simulink model "mpc_psm"  (R2026b)
settings: Solver=ode23tb  StopTime=param.sim.simlength  FixedStep=param.glb_time.tc  MaxStep=param.glb_time.tc
values from neighbouring files (symbols this model uses):
  param = struct()    [init_model.m]
undefined symbols (not defined in the file or in its folder): tc
libraries: fl_lib x28, nesl_utility x13, cstblocks_lti x6, lithium_ion_battery x1, dclink_with_center_tap x1, ideal_bridges_lib x1, dead_time_generator_cmos_simulink x1, single_phase_pwm_modulator x1, threephase_inductor_lib x1, simple_flexible_shaft x1, permanent_magnet_synchronous_machine x1
(part 3 of 3)

== system mpc_psm/inv_psm_mod1/inverter_ctrl/inverter_control/phase_compensation_1/alignment_ctrl/pi ==
  u_ref : Inport
  u : Inport  Port=2
  1/Ti : Gain  Gain=kp  SaturateOnIntegerOverflow=on  OutDataTypeStr=Inherit: Same as input  ParamDataTypeStr=Inherit: Same as input
  Saturation : Saturate  UpperLimit=lim_up  LowerLimit=lim_down
  Sum1 : Sum  Inputs=+++  SaturateOnIntegerOverflow=on
  Sum2 : Sum  Inputs=-+  SaturateOnIntegerOverflow=on
  Sum3 : Sum  Inputs=-+  SaturateOnIntegerOverflow=on
  Unit Delay4 : UnitDelay  SampleTime=-1
  kp : Gain  Gain=ki  SaturateOnIntegerOverflow=on  OutDataTypeStr=Inherit: Same as input  ParamDataTypeStr=Inherit: Same as input
  y : Outport
  wires:
  1/Ti/1 -> Sum1/1, Sum3/1
  kp/1 -> Sum1/2
  Sum3/1 -> Unit Delay4/1
  Unit Delay4/1 -> Sum1/3
  u_ref/1 -> Sum2/2
  u/1 -> Sum2/1
  Sum2/1 -> kp/1, 1/Ti/1
  Sum1/1 -> Saturation/1
  Saturation/1 -> Sum3/2, y/1

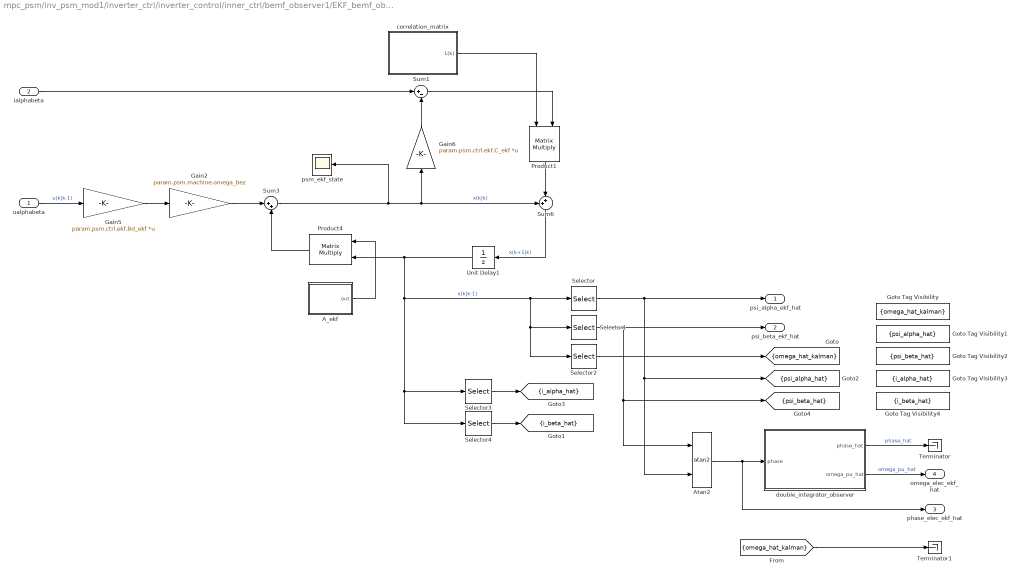
== system mpc_psm/inv_psm_mod1/inverter_ctrl/inverter_control/inner_ctrl/bemf_observer1/EKF_bemf_observer/extended_kalman_observer ==
  ualphabeta : Inport
  ialphabeta : Inport  Port=2
  A_ekf : Subsystem
  Atan2 : Trigonometry  Operator=atan2
  Gain2 : Gain  Gain=param.psm.machine.omega_bez
  Gain5 : Gain  Gain=param.psm.ctrl.ekf.Bd_ekf  Multiplication=Matrix(K*u)
  Gain6 : Gain  Gain=param.psm.ctrl.ekf.C_ekf  Multiplication=Matrix(K*u)
  Goto Tag Visibility : GotoTagVisibility  GotoTag=omega_hat_kalman
  Goto Tag Visibility1 : GotoTagVisibility  GotoTag=psi_alpha_hat
  Goto Tag Visibility2 : GotoTagVisibility  GotoTag=psi_beta_hat
  Goto Tag Visibility3 : GotoTagVisibility  GotoTag=i_alpha_hat
  Goto Tag Visibility4 : GotoTagVisibility  GotoTag=i_beta_hat
  Product1 : Product  Multiplication=Matrix(*)
  Product4 : Product  Multiplication=Matrix(*)
  Selector : Selector  InputPortWidth=6  IndexOptions=Index vector (dialog)  Indices=3  OutputSizes=1  RuntimeRangeChecks=off
  Selector1 : Selector  InputPortWidth=6  IndexOptions=Index vector (dialog)  Indices=4  OutputSizes=1  RuntimeRangeChecks=off
  Selector2 : Selector  InputPortWidth=6  IndexOptions=Index vector (dialog)  Indices=5  OutputSizes=1  RuntimeRangeChecks=off
  Selector3 : Selector  InputPortWidth=6  IndexOptions=Index vector (dialog)  Indices=1  OutputSizes=1  RuntimeRangeChecks=off
  Selector4 : Selector  InputPortWidth=6  IndexOptions=Index vector (dialog)  Indices=2  OutputSizes=1  RuntimeRangeChecks=off
  Sum1 : Sum  Inputs=|+-
  Sum3 : Sum  Inputs=|++
  Sum6 : Sum  Inputs=++|
  Terminator : Terminator
  Terminator1 : Terminator
  Unit Delay1 : UnitDelay  InitialCondition=[0 0 1 1 0 0]*param.glb_time.ts_inv  SampleTime=-1
  correlation_matrix : Subsystem
  double_integrator_observer : Subsystem
  psm_ekf_state : Scope
      settings: ActiveDisplayYMinimum=-2.6651275002473325  ActiveDisplayYMaximum=3.9005956712949552
  psi_alpha_ekf_hat : Outport
  psi_beta_ekf_hat : Outport  Port=2
  phase_elec_ekf_hat : Outport  Port=3
  omega_elec_ekf_hat : Outport  Port=4
  tag scope: i_alpha_hat=scoped, i_beta_hat=scoped, omega_hat_kalman=scoped, psi_alpha_hat=scoped, psi_beta_hat=scoped
  wires:
  Gain5/1 -> Gain2/1
  Gain6/1 -> Sum1/2
  Sum6/1 -> Unit Delay1/1  "x(k+1|k)"
  Sum1/1 -> Product1/2
  ialphabeta/1 -> Sum1/1
  ualphabeta/1 -> Gain5/1  "u(k|k-1)"
  Sum3/1 -> psm_ekf_state/1, Gain6/1, Sum6/1  "x(k|k)"
  Unit Delay1/1 -> Selector2/1, Selector1/1, Selector/1, Selector3/1, Selector4/1, Product4/2  "x(k|k-1)"
  A_ekf/1(out) -> Product4/1
  Selector1/1 -> Atan2/1, [psi_beta_hat], psi_beta_ekf_hat/1
  Selector/1 -> Atan2/2, [psi_alpha_hat], psi_alpha_ekf_hat/1
  Selector2/1 -> [omega_hat_kalman]
  Selector3/1 -> [i_alpha_hat]
  Selector4/1 -> [i_beta_hat]
  Product4/1 -> Sum3/2
  Atan2/1 -> phase_elec_ekf_hat/1, double_integrator_observer/1(phase)
  Gain2/1 -> Sum3/1
  Product1/1 -> Sum6/2
  correlation_matrix/1(L(k)) -> Product1/1
  double_integrator_observer/1(phase_hat) -> Terminator/1  "phase_hat"
  double_integrator_observer/2(omega_pu_hat) -> omega_elec_ekf_hat/1  "omega_pu_hat"
  [omega_hat_kalman] -> Terminator1/1

== system mpc_psm/inv_psm_mod1/inverter_ctrl/inverter_control/inner_ctrl/bemf_observer1/bemf_observer/double_integrator_observer ==
  theta : Inport
  Dead Zone : DeadZone  LowerValue=-0.01  UpperValue=0.01
  Gain : Gain  Gain=param.psm.ctrl.di_obs.komega
  Gain1 : Gain  Gain=param.psm.ctrl.di_obs.ktheta
  Gain2 : Gain  Gain=param.psm.machine.omega_bez
  Gain3 : Gain  Gain=1/param.psm.machine.omega_bez
  Gain4 : Gain  Gain=param.glb_time.ts_inv
  Gain5 : Gain  Gain=param.glb_time.ts_inv
  Gain6 : Gain  Gain=param.glb_time.ts_inv
  Sum : Sum  Inputs=-+|
  Sum1 : Sum  Inputs=|++
  Sum2 : Sum  Inputs=|++
  Sum8 : Sum  Inputs=++|
  Unit Delay1 : UnitDelay  InitialCondition=pi  SampleTime=-1
  Unit Delay2 : UnitDelay  SampleTime=-1
  bounder1 : MATLAB Function  TreatAsAtomicUnit=on
  bounder2 : MATLAB Function  TreatAsAtomicUnit=on
  omega_pu_hat : Outport  VectorParamsAs1DForOutWhenUnconnected=off
  theta_hat : Outport  Port=2  VectorParamsAs1DForOutWhenUnconnected=off
  wires:
  Gain1/1 -> Gain6/1
  theta/1 -> Sum/2  "theta_bemf"
  Sum8/1 -> Unit Delay1/1
  Unit Delay1/1 -> bounder2/1(u)
  Sum1/1 -> Unit Delay2/1
  Gain/1 -> Gain4/1
  Unit Delay2/1 -> omega_pu_hat/1, Sum1/2, Gain5/1
  Sum2/1 -> Sum8/2
  bounder2/1(y) -> Sum2/2, theta_hat/1, Sum/1  "theta_hat"
  bounder1/1(y) -> Gain1/1, Gain/1
  Gain2/1 -> Sum8/1
  Gain3/1 -> Sum1/1
  Gain5/1 -> Gain2/1
  Sum/1 -> bounder1/1(u)
  Gain4/1 -> Gain3/1
  Gain6/1 -> Sum2/1

== system mpc_psm/inv_psm_mod1/inverter_ctrl/inverter_control/inner_ctrl/bemf_observer1/bemf_observer/psi_alpha_hat ==
  ualpha : Inport
  ialpha : Inport  Port=2
  udc : Inport  Port=3
  Gain1 : Gain  Gain=param.psm.ctrl.mpc.R_norm
  Gain2 : Gain  Gain=param.psm.ctrl.emf_fb_p
  Gain3 : Gain  Gain=param.psm.ctrl.emf_p
  Gain4 : Gain  Gain=param.psm.machine.omega_bez
  Gain5 : Gain  Gain=param.psm.ctrl.mpc.L_norm
  Gain6 : Gain  Gain=param.psm.ctrl.u_psm_scale
  Gain7 : Gain  Gain=param.glb_time.ts_inv
  Product : Product  RndMeth=Zero
  Sum : Sum  Inputs=|+-
  Sum1 : Sum  Inputs=|+-
  Sum2 : Sum  Inputs=++-  SaturateOnIntegerOverflow=on
  Sum3 : Sum  Inputs=|++
  Sum4 : Sum  Inputs=+-  SaturateOnIntegerOverflow=on
  Unit Delay1 : UnitDelay  SampleTime=-1
  Unit Delay2 : UnitDelay  SampleTime=-1
  Unit Delay3 : UnitDelay  SampleTime=-1
  psi_s_alpha_hat : Outport  VectorParamsAs1DForOutWhenUnconnected=off
  psi_r_alpha_hat : Outport  Port=2  VectorParamsAs1DForOutWhenUnconnected=off
  wires:
  [psi_r_m_alpha_mod1] -> Sum1/1
  [psi_r_alpha_hat_mod1] -> Sum1/2
  Gain4/1 -> Gain7/1
  Sum2/1 -> Gain4/1
  Gain3/1 -> Sum2/3
  ialpha/1 -> Gain5/1, Gain1/1
  Gain1/1 -> Sum/2
  Sum/1 -> Sum2/2
  ualpha/1 -> Product/1
  Gain5/1 -> Unit Delay3/1
  Unit Delay1/1 -> Sum4/1, psi_s_alpha_hat/1, Gain3/1, Sum3/2
  Sum3/1 -> Unit Delay1/1
  Sum4/1 -> Unit Delay2/1
  Sum1/1 -> Gain2/1
  Gain2/1 -> Sum2/1
  Gain7/1 -> Sum3/1
  Product/1 -> Gain6/1
  Gain6/1 -> Sum/1
  Unit Delay2/1 -> psi_r_alpha_hat/1
  Unit Delay3/1 -> Sum4/2
  udc/1 -> Product/2

== system mpc_psm/inv_psm_mod1/inverter_ctrl/inverter_control/inner_ctrl/bemf_observer1/bemf_observer/psi_beta_hat ==
  ubeta : Inport
  ibeta : Inport  Port=2
  udc : Inport  Port=3
  Gain1 : Gain  Gain=param.psm.ctrl.mpc.R_norm
  Gain2 : Gain  Gain=param.psm.ctrl.emf_fb_p
  Gain3 : Gain  Gain=param.psm.ctrl.emf_p
  Gain4 : Gain  Gain=param.psm.machine.omega_bez
  Gain5 : Gain  Gain=param.psm.ctrl.mpc.L_norm
  Gain6 : Gain  Gain=param.psm.ctrl.u_psm_scale
  Gain7 : Gain  Gain=param.glb_time.ts_inv
  Product : Product  RndMeth=Zero
  Sum : Sum  Inputs=|+-
  Sum1 : Sum  Inputs=|+-
  Sum2 : Sum  Inputs=++-  SaturateOnIntegerOverflow=on
  Sum3 : Sum  Inputs=|++
  Sum4 : Sum  Inputs=+-  SaturateOnIntegerOverflow=on
  Unit Delay1 : UnitDelay  SampleTime=-1
  Unit Delay2 : UnitDelay  SampleTime=-1
  Unit Delay3 : UnitDelay  SampleTime=-1
  psi_s_beta_hat : Outport  VectorParamsAs1DForOutWhenUnconnected=off
  psi_r_beta_hat : Outport  Port=2  VectorParamsAs1DForOutWhenUnconnected=off
  wires:
  Gain5/1 -> Unit Delay3/1
  Sum/1 -> Sum2/2
  Gain1/1 -> Sum/2
  ibeta/1 -> Gain5/1, Gain1/1
  Gain3/1 -> Sum2/3
  Sum2/1 -> Gain4/1
  Gain4/1 -> Gain7/1
  Sum1/1 -> Gain2/1
  [psi_r_beta_hat_mod1] -> Sum1/2
  [psi_r_m_beta_mod1] -> Sum1/1
  Unit Delay1/1 -> Gain3/1, Sum4/1, psi_s_beta_hat/1, Sum3/2
  Sum3/1 -> Unit Delay1/1
  Sum4/1 -> Unit Delay2/1
  Gain2/1 -> Sum2/1
  ubeta/1 -> Product/1
  Gain7/1 -> Sum3/1
  Product/1 -> Gain6/1
  Gain6/1 -> Sum/1
  Unit Delay2/1 -> psi_r_beta_hat/1
  Unit Delay3/1 -> Sum4/2
  udc/1 -> Product/2

== system mpc_psm/inv_psm_mod1/inverter_ctrl/inverter_control/inner_ctrl/bemf_observer1/bemf_observer/theta_bemf_hat ==
  psi_r_alpha_hat : Inport
  psi_r_beta_hat : Inport  Port=2
  Trigonometric Function : Trigonometry  Operator=atan2  OutputSignalType=real
  theta_emf_hat : Outport  VectorParamsAs1DForOutWhenUnconnected=off
  wires:
  psi_r_alpha_hat/1 -> Trigonometric Function/2
  psi_r_beta_hat/1 -> Trigonometric Function/1
  Trigonometric Function/1 -> theta_emf_hat/1

== system mpc_psm/inv_psm_mod1/inverter_ctrl/inverter_control/inner_ctrl/bemf_observer1/bemf_observer_ccaller/Reset Trigger ==
  Step : Step  Time=0.01  InitialValue=1  FinalValue=0
  Out1 : Outport
  wires:
  Step/1 -> Out1/1  "Reset"

== system mpc_psm/inv_psm_mod1/inverter_ctrl/inverter_control/inner_ctrl/bemf_observer1/EKF_bemf_observer/extended_kalman_observer/A_ekf ==
  Gain1 : Gain  Gain=param.psm.ctrl.ekf.A6_pred_ekf
  Gain{7,9..10,13,20} (5 alike) : Gain  Gain=param.psm.machine.omega_bez
  Gain{2,4,6,11,16,18} (6 alike) : Gain  Gain=param.glb_time.ts_inv
  Gain15 : Gain  Gain=param.psm.ctrl.ekf.A2_tilde_ekf
  Gain17 : Gain  Gain=param.psm.ctrl.ekf.A3_tilde_ekf
  Gain3 : Gain  Gain=param.psm.ctrl.ekf.A4_tilde_ekf
  Gain5 : Gain  Gain=param.psm.ctrl.ekf.A5_tilde_ekf
  I1 : Constant  Value=eye(6)
  I2 : Constant  Value=param.psm.ctrl.ekf.A1_tilde_ekf
  Sum7 : Sum  Inputs=+++++++
  out : Outport
  wires:
  Sum7/1 -> out/1
  I2/1 -> Gain11/1
  I1/1 -> Sum7/1
  Gain1/1 -> Gain2/1
  Gain3/1 -> Gain4/1
  Gain5/1 -> Gain6/1
  [omega_hat_kalman] -> Gain1/1
  [psi_alpha_hat] -> Gain3/1
  [psi_beta_hat] -> Gain5/1
  Gain11/1 -> Gain7/1
  Gain4/1 -> Gain9/1
  Gain6/1 -> Gain10/1
  Gain7/1 -> Sum7/2
  Gain9/1 -> Sum7/5
  Gain10/1 -> Sum7/6
  Gain18/1 -> Gain13/1
  Gain16/1 -> Gain20/1
  Gain17/1 -> Gain18/1
  Gain15/1 -> Gain16/1
  Gain13/1 -> Sum7/4
  Gain20/1 -> Sum7/3
  [i_beta_hat] -> Gain17/1
  [i_alpha_hat] -> Gain15/1
  Gain2/1 -> Sum7/7

== system mpc_psm/inv_psm_mod1/inverter_ctrl/inverter_control/inner_ctrl/bemf_observer1/EKF_bemf_observer/extended_kalman_observer/correlation_matrix ==
  A_ekf : Subsystem
  Gain1 : Gain  Gain=param.psm.ctrl.ekf.C_ekf  Multiplication=Matrix(u*K)
  Gain10 : Gain  Gain=param.psm.ctrl.ekf.C_ekf'  Multiplication=Matrix(u*K)
  Gain8 : Gain  Gain=param.psm.ctrl.ekf.C_ekf'  Multiplication=Matrix(u*K)
  Gain9 : Gain  Gain=param.psm.ctrl.ekf.C_ekf  Multiplication=Matrix(K*u)
  I6 : Constant  Value=eye(6)
  Product{,2,5..6} (4 alike) : Product  Multiplication=Matrix(*)
  Product3 : Product  Inputs=*/  Multiplication=Matrix(*)
  Q : Constant  Value=param.psm.ctrl.ekf.Qkalman
  R : Constant  Value=param.psm.ctrl.ekf.Rkalman
  R1 : Constant  Value=eye(2)
  Sum2 : Sum  Inputs=+-|
  Sum4 : Sum  Inputs=|++
  Sum5 : Sum  Inputs=|++
  Transpose : Math  Operator=transpose
  Unit Delay2 : UnitDelay  SampleTime=-1
  L(k) : Outport
  wires:
  A_ekf/1(out) -> Transpose/1, Product5/1
  Product6/1 -> Sum5/1
  Product3/1 -> Product/2
  Gain8/1 -> Product/1
  Sum4/1 -> Product3/2
  Sum5/1 -> Gain8/1, Gain9/1, Product2/2  "P(k|k)"
  Sum2/1 -> Product2/1
  Product/1 -> Gain1/1, L(k)/1  "L(k)"
  Gain1/1 -> Sum2/2
  R1/1 -> Product3/1
  Product2/1 -> Unit Delay2/1  "P(k+1|k)"
  Product5/1 -> Product6/1
  Gain10/1 -> Sum4/1
  Transpose/1 -> Product6/2
  R/1 -> Sum4/2
  Q/1 -> Sum5/2
  Unit Delay2/1 -> Product5/2
  Gain9/1 -> Gain10/1
  I6/1 -> Sum2/1

== system mpc_psm/inv_psm_mod1/inverter_ctrl/inverter_control/inner_ctrl/bemf_observer1/EKF_bemf_observer/extended_kalman_observer/double_integrator_observer ==
  phase : Inport
  Gain : Gain  Gain=param.psm.ctrl.di_obs.komega
  Gain1 : Gain  Gain=param.psm.ctrl.di_obs.ktheta
  Gain2 : Gain  Gain=param.psm.machine.omega_bez
  Gain3 : Gain  Gain=1/param.psm.machine.omega_bez
  Gain4 : Gain  Gain=param.glb_time.ts_inv
  Gain5 : Gain  Gain=param.glb_time.ts_inv
  Gain6 : Gain  Gain=param.glb_time.ts_inv
  Sum : Sum  Inputs=-+|
  Sum1 : Sum  Inputs=|++
  Sum2 : Sum  Inputs=|++
  Sum8 : Sum  Inputs=++|
  Unit Delay1 : UnitDelay  InitialCondition=pi  SampleTime=-1
  Unit Delay2 : UnitDelay  SampleTime=-1
  bounder1 : MATLAB Function  TreatAsAtomicUnit=on
  bounder2 : MATLAB Function  TreatAsAtomicUnit=on
  phase_hat : Outport  VectorParamsAs1DForOutWhenUnconnected=off
  omega_pu_hat : Outport  Port=2  VectorParamsAs1DForOutWhenUnconnected=off
  wires:
  Gain1/1 -> Gain6/1
  phase/1 -> Sum/2
  Sum8/1 -> Unit Delay1/1
  Unit Delay1/1 -> bounder2/1(u)
  Sum1/1 -> Unit Delay2/1
  Gain/1 -> Gain4/1
  Unit Delay2/1 -> omega_pu_hat/1, Sum1/2, Gain5/1
  Sum2/1 -> Sum8/2
  bounder2/1(y) -> Sum2/2, phase_hat/1, Sum/1  "phase_hat"
  bounder1/1(y) -> Gain/1, Gain1/1
  Gain2/1 -> Sum8/1
  Gain3/1 -> Sum1/1
  Gain5/1 -> Gain2/1
  Sum/1 -> bounder1/1(u)
  Gain4/1 -> Gain3/1
  Gain6/1 -> Sum2/1

== system mpc_psm/inv_psm_mod1/inverter_ctrl/inverter_control/inner_ctrl/bemf_observer1/EKF_bemf_observer/extended_kalman_observer/correlation_matrix/A_ekf ==
  Gain1 : Gain  Gain=param.psm.ctrl.ekf.A6_tilde_ekf
  Gain{7..10,13,20} (6 alike) : Gain  Gain=param.psm.machine.omega_bez
  Gain{2,4,6,11,16,18} (6 alike) : Gain  Gain=param.glb_time.ts_inv
  Gain15 : Gain  Gain=param.psm.ctrl.ekf.A2_tilde_ekf
  Gain17 : Gain  Gain=param.psm.ctrl.ekf.A3_tilde_ekf
  Gain3 : Gain  Gain=param.psm.ctrl.ekf.A4_tilde_ekf
  Gain5 : Gain  Gain=param.psm.ctrl.ekf.A5_tilde_ekf
  I1 : Constant  Value=eye(6)
  I2 : Constant  Value=param.psm.ctrl.ekf.A1_tilde_ekf
  Sum7 : Sum  Inputs=+++++++
  out : Outport
  wires:
  Sum7/1 -> out/1
  I2/1 -> Gain11/1
  I1/1 -> Sum7/1
  Gain1/1 -> Gain2/1
  Gain3/1 -> Gain4/1
  Gain5/1 -> Gain6/1
  [omega_hat_kalman] -> Gain1/1
  [psi_alpha_hat] -> Gain3/1
  [psi_beta_hat] -> Gain5/1
  Gain11/1 -> Gain7/1
  Gain2/1 -> Gain8/1
  Gain4/1 -> Gain9/1
  Gain6/1 -> Gain10/1
  Gain7/1 -> Sum7/2
  Gain9/1 -> Sum7/5
  Gain10/1 -> Sum7/6
  Gain8/1 -> Sum7/7
  Gain18/1 -> Gain13/1
  Gain16/1 -> Gain20/1
  Gain17/1 -> Gain18/1
  Gain15/1 -> Gain16/1
  Gain13/1 -> Sum7/4
  Gain20/1 -> Sum7/3
  [i_beta_hat] -> Gain17/1
  [i_alpha_hat] -> Gain15/1

== matlab function mpc_psm/inv_psm_mod1/inverter_ctrl/inverter_control/inner_ctrl/bemf_observer1/bemf_observer/double_integrator_observer/bounder1 ==
  data: u input; y output
function y = bounder(u)
    
    y = -pi + mod(u+3*pi,2*pi);
end

== matlab function mpc_psm/inv_psm_mod1/inverter_ctrl/inverter_control/inner_ctrl/current_transformation/uvw2alphabeta ==
  data: u input; alpha output; v input; w input; beta output
function [alpha,beta] = uvw2alphabeta(u,v,w)

alpha = 2/3*(u - 1/2*v - 1/2*w);
beta  = 2/3*(sqrt(3)/2*(v - w));

end

== matlab function mpc_psm/inv_psm_mod1/inverter_ctrl/inverter_control/inner_ctrl/bemf_observer1/bemf_observer/double_integrator_observer/bounder2 ==
  data: u input; y output
function y = bounder(u)
    
    u = -pi + mod(u+3*pi,2*pi);
    
    y = u;
end

== matlab function mpc_psm/inv_psm_mod1/inverter_ctrl/inverter_control/inner_ctrl/bemf_observer1/EKF_bemf_observer/extended_kalman_observer/double_integrator_observer/bounder2 ==
  data: u input; y output
function y = bounder(u)
    y = -pi + mod(u+3*pi,2*pi);
end

== matlab function mpc_psm/inv_psm_mod1/inverter/inverter/timer/MATLAB Function ==
  data: t input; y output; phase input; period input
function y = ramp_up_down(t,phase,period)
x = sin(2*pi/period*t - phase -pi/2);
y = asin(x)/pi + 1/2;

== matlab function mpc_psm/inv_psm_mod1/inverter_ctrl/inverter_control/encoder-sensorless-switch/double_integrator_observer/bounder1 ==
  data: u input; y output
function y = bounder(u)
    y = -pi + mod(u+3*pi,2*pi);
end

== matlab function mpc_psm/inv_psm_mod1/inverter_ctrl/inverter_control/encoder-sensorless-switch/double_integrator_observer/bounder2 ==
  data: u input; y output
function y = bounder(u)
    y = -pi + mod(u+3*pi,2*pi);
end

== matlab function mpc_psm/inv_psm_mod1/inverter_ctrl/inverter_control/inner_ctrl/bemf_observer1/EKF_bemf_observer/extended_kalman_observer/double_integrator_observer/bounder1 ==
  data: u input; y output
function y = bounder(u)
    y = -pi + mod(u+3*pi,2*pi);
end

== matlab function mpc_psm/inv_psm_mod1/inverter_ctrl/inverter_control/inner_ctrl/mp control/mpc_pu_d ==
  data: vdc input; ialpha_ref input; ibeta_ref input; ialpha input; ualpha output; ibeta input; omega_hat input; psi_alpha_hat input; psi_beta_hat input; ubeta output; cmg_g1 output; cmg_g2 output; cmg_g3 output; cmg_g4 output; cmg_g5 output; cmg_g6 output; u_scale input; L_norm input; omega_bez input; R_norm input; k_kalman input; k_sw input; ts_inv input
function [ualpha, ubeta, cmg_g1, cmg_g2, cmg_g3, cmg_g4, cmg_g5, cmg_g6] = mpc(vdc, ialpha_ref, ...
    ibeta_ref, ialpha, ibeta, omega_hat, psi_alpha_hat, psi_beta_hat, u_scale, ...
    L_norm, omega_bez, R_norm, k_kalman, k_sw, ts_inv)
% Finite-set predictive current control of the two-level bridge: every control step it tests the 8 states
% of the bridge and applies the one with the lowest cost (current error and switching).
%
% Inputs, all per unit of the machine:
%   vdc                     DC-link voltage measured one control step before, pu of udc_nom
%   ialpha_ref, ibeta_ref   current reference, pu of ibez
%   ialpha, ibeta           current measured one control step before, pu of ibez
%   omega_hat               speed of the EKF block, pu of omega_bez
%   psi_alpha_hat, psi_beta_hat   flux of the EKF, pu of psi_m
%   u_scale                 udc_nom/ubez: voltage in pu of udc_nom -> voltage in pu of ubez
%   L_norm, R_norm          inductance and resistance seen by the bridge: q axis of the machine plus the output
%                           inductor, pu of the machine (the EKF uses the same values)
%   omega_bez               [rad/s] electrical base pulsation
%   k_kalman, k_sw          weights of the current error and of the number of legs that change state
%   ts_inv                  [s] control step
% Outputs:
%   ualpha, ubeta           voltage of the vector applied in the last step, pu of ubez. The Unit Delay after
%                           this block makes it the vector of two steps before: the vector that acted before the
%                           current measured one step before, the pair the EKF needs.
%   cmg_g1 ... cmg_g6       gate commands (0 or 15 V) of a+, a-, b+, b-, c+, c- (the dead time is added in
%                           the inverter by the gate generator)
%
% Timing: current and DC voltage are measured one control step before, and the vector chosen now acts until
% the next step. So the control first computes the current of now with the vector of the last step (delay
% compensation), then chooses the vector for the next step.

    persistent states_table u_last s_last

    if isempty(states_table)
        % the 8 states [leg a, leg b, leg c]: 1 = upper switch on, 0 = lower switch on
        states_table = [0 0 0; 1 0 0; 1 1 0; 0 1 0; 0 1 1; 0 0 1; 1 0 1; 1 1 1];
        u_last = [0; 0];            % voltage of the vector applied in the last step, pu of ubez
        s_last = [0 0 0];           % legs of the vector applied in the last step
    end

    Vdd = 15;
    inv_sqrt3 = 0.577350269189626;
    ts_pu = ts_inv*omega_bez;
    g = ts_pu/L_norm;

    % back-EMF of the EKF flux, e = d(psi)/dt = j*omega*psi (pu of ubez)
    ealpha = -omega_hat*psi_beta_hat;
    ebeta = omega_hat*psi_alpha_hat;

    % 1. Delay compensation: current of now, from the current measured one step before and the vector
    %    applied since then
    ialpha0 = ialpha + g*(u_last(1) - R_norm*ialpha - ealpha);
    ibeta0 = ibeta + g*(u_last(2) - R_norm*ibeta - ebeta);

    % 2. Prediction and cost of the 8 states (the first state with the lowest cost wins)
    minJ = 1e18;
    best_idx = 1;
    ua_best = 0.0;
    ub_best = 0.0;

    for n = 1:8
        sa = states_table(n,1);
        sb = states_table(n,2);
        sc = states_table(n,3);

        % alpha/beta voltage of the state, pu of ubez (leg voltages sa*vdc, sb*vdc, sc*vdc)
        ua = u_scale*vdc*(sa - 0.5*sb - 0.5*sc)*2/3;
        ub = u_scale*vdc*(sb - sc)*inv_sqrt3;

        % current at the next step
        ia_p = ialpha0 + g*(ua - R_norm*ialpha0 - ealpha);
        ib_p = ibeta0 + g*(ub - R_norm*ibeta0 - ebeta);

        % legs that change state from the vector of the last step
        nsw = abs(sa - s_last(1)) + abs(sb - s_last(2)) + abs(sc - s_last(3));

        % cost
        J = k_kalman*((ialpha_ref - ia_p)^2 + (ibeta_ref - ib_p)^2) + k_sw*nsw;

        if J < minJ
            minJ = J;
            best_idx = n;
            ua_best = ua;
            ub_best = ub;
        end
    end

    % 3. Voltage for the observers (vector of the last step), then the memory of the applied vector
    ualpha = u_last(1);
    ubeta = u_last(2);
    u_last = [ua_best; ub_best];
    s_last = states_table(best_idx, :);

    % 4. Gate commands of the chosen state
    ga = states_table(best_idx, 1);
    gb = states_table(best_idx, 2);
    gc = states_table(best_idx, 3);

    cmg_g1 = Vdd*ga;
    cmg_g2 = Vdd*(1 - ga);
    cmg_g3 = Vdd*gb;
    cmg_g4 = Vdd*(1 - gb);
    cmg_g5 = Vdd*gc;
    cmg_g6 = Vdd*(1 - gc);
end

== matlab function mpc_psm/inv_psm_mod1/inverter_ctrl/inverter_control/encoder-sensorless-switch/MATLAB Function ==
  data: omega_psm input; omega_ctrl output; phase_psm input; omega_obs input; phase_obs input; phase_ctrl output; omega_th input
function [omega_ctrl, phase_ctrl] = switch_enc2obs(omega_psm, phase_psm, omega_obs, phase_obs, omega_th)

if abs(omega_psm) > omega_th
    omega_ctrl = omega_obs;
    phase_ctrl = phase_obs;
else
    omega_ctrl = omega_psm;
    phase_ctrl = phase_psm;
end

== matlab function mpc_psm/inv_psm_mod1/inverter_ctrl/inverter_control/inner_ctrl/current_transformation/alphabeta2dq ==
  data: alpha input; d output; beta input; gamma input; q output
function [d,q] = alphabeta2dq(alpha,beta,gamma)

    d  =  alpha*cos(gamma) + beta*sin(gamma);
    q = -alpha*sin(gamma) + beta*cos(gamma);

end
